simulink model "fw_watchdog_mgr"  (R2026b)
settings: Solver=VariableStepAuto
undefined symbols (not defined in the file or in its folder): DiscIntNeverNeededParam, P, ShaddadMode, Ts
libraries: simulink x10
settings Model: Creator=aomar  LastModifiedBy=aomar

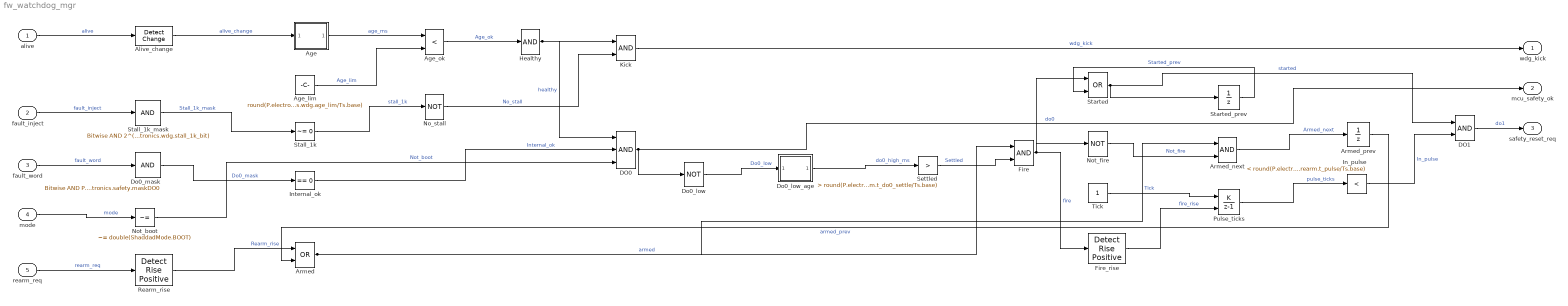
== system fw_watchdog_mgr ==
  alive : Inport  OutDataTypeStr=uint8  PortDimensions=3  SampleTime=Ts.base
  fault_inject : Inport  Port=2  OutDataTypeStr=uint32  SampleTime=Ts.base
  fault_word : Inport  Port=3  OutDataTypeStr=uint32  SampleTime=Ts.base
  mode : Inport  Port=4  OutDataTypeStr=uint8  SampleTime=Ts.base
  rearm_req : Inport  Port=5  OutDataTypeStr=boolean  SampleTime=Ts.base
  Age : Subsystem
  Age_lim : Constant  Value=round(P.electronics.wdg.age_lim/Ts.base)  OutDataTypeStr=uint16  SampleTime=Ts.base
  Age_ok : RelationalOperator  Operator=<  OutDataTypeStr=boolean  RndMeth=Simplest  InputSameDT=off
  Alive_change : simulink/Logic and Bit Operations/Detect Change  vinit=0  OutDataTypeStr=boolean
  Armed : Logic  Operator=OR  AllPortsSameDT=off  OutDataTypeStr=boolean
  Armed_next : Logic  AllPortsSameDT=off  OutDataTypeStr=boolean
  Armed_prev : UnitDelay  InitialCondition=false  SampleTime=-1
  DO0 : Logic  Inputs=3  AllPortsSameDT=off  OutDataTypeStr=boolean
  DO1 : Logic  AllPortsSameDT=off  OutDataTypeStr=boolean
  Do0_low : Logic  Operator=NOT  Inputs=1  AllPortsSameDT=off  OutDataTypeStr=boolean
  Do0_low_age : Subsystem
  Do0_mask : simulink/Logic and Bit Operations/Bitwise Operator  logicop=AND  UseBitMask=on  BitMask=P.electronics.safety.maskDO0  BitMaskRealWorld=Stored Integer
  Fire : Logic  AllPortsSameDT=off  OutDataTypeStr=boolean
  Fire_rise : simulink/Logic and Bit Operations/Detect Rise Positive  vinit=0  OutDataTypeStr=boolean
  Healthy : Logic  Inputs=1  AllPortsSameDT=off  OutDataTypeStr=boolean
  In_pulse : simulink/Logic and Bit Operations/Compare To Constant  relop=<  const=round(P.electronics.safety.rearm.t_pulse/Ts.base)  OutDataTypeStr=boolean
  Internal_ok : simulink/Logic and Bit Operations/Compare To Zero  relop===  OutDataTypeStr=boolean
  Kick : Logic  AllPortsSameDT=off  OutDataTypeStr=boolean
  No_stall : Logic  Operator=NOT  Inputs=1  AllPortsSameDT=off  OutDataTypeStr=boolean
  Not_boot : simulink/Logic and Bit Operations/Compare To Constant  relop=~=  const=double(ShaddadMode.BOOT)  OutDataTypeStr=boolean
  Not_fire : Logic  Operator=NOT  Inputs=1  AllPortsSameDT=off  OutDataTypeStr=boolean
  Pulse_ticks : DiscreteIntegrator  IntegratorMethod=Accumulation: Forward Euler  ExternalReset=rising  SampleTime=-1  OutDataTypeStr=single  LimitOutput=on  UpperSaturationLimit=round(P.electronics.safety.rearm.t_pulse/Ts.base) + 1  LowerSaturationLimit=0  ICPrevOutput=DiscIntNeverNeededParam  ICPrevScaledInput=DiscIntNeverNeededParam
  Rearm_rise : simulink/Logic and Bit Operations/Detect Rise Positive  vinit=0  OutDataTypeStr=boolean
  Settled : simulink/Logic and Bit Operations/Compare To Constant  relop=>  const=round(P.electronics.safety.rearm.t_do0_settle/Ts.base)  OutDataTypeStr=boolean
  Stall_1k : simulink/Logic and Bit Operations/Compare To Zero  relop=~=  OutDataTypeStr=boolean
  Stall_1k_mask : simulink/Logic and Bit Operations/Bitwise Operator  logicop=AND  UseBitMask=on  BitMask=2^(P.electronics.wdg.stall_1k_bit)  BitMaskRealWorld=Stored Integer
  Started : Logic  Operator=OR  AllPortsSameDT=off  OutDataTypeStr=boolean
  Started_prev : UnitDelay  InitialCondition=false  SampleTime=-1
  Tick : Constant  OutDataTypeStr=single  SampleTime=Ts.base
  wdg_kick : Outport  OutDataTypeStr=boolean
  mcu_safety_ok : Outport  Port=2  OutDataTypeStr=boolean
  safety_reset_req : Outport  Port=3  OutDataTypeStr=boolean
  wires:
  alive/1 -> Alive_change/1  "alive"
  fault_inject/1 -> Stall_1k_mask/1  "fault_inject"
  fault_word/1 -> Do0_mask/1  "fault_word"
  mode/1 -> Not_boot/1  "mode"
  rearm_req/1 -> Rearm_rise/1  "rearm_req"
  Not_boot/1 -> DO0/3  "Not_boot"
  Stall_1k_mask/1 -> Stall_1k/1  "Stall_1k_mask"
  Do0_mask/1 -> Internal_ok/1  "Do0_mask"
  Alive_change/1 -> Age/1(fresh)  "alive_change"
  Rearm_rise/1 -> Armed/1  "Rearm_rise"
  Age_lim/1 -> Age_ok/2  "Age_lim"
  Stall_1k/1 -> No_stall/1  "stall_1k"
  Internal_ok/1 -> DO0/2  "Internal_ok"
  Armed/1 -> Armed_next/1, Fire/1  "armed"
  Age/1(ticks) -> Age_ok/1  "age_ms"
  Age_ok/1 -> Healthy/1  "Age_ok"
  No_stall/1 -> Kick/2  "No_stall"
  Healthy/1 -> DO0/1, Kick/1  "healthy"
  Kick/1 -> wdg_kick/1  "wdg_kick"
  DO0/1 -> mcu_safety_ok/1, Do0_low/1  "do0"
  Do0_low/1 -> Do0_low_age/1(fresh)  "Do0_low"
  Do0_low_age/1(ticks) -> Settled/1  "do0_high_ms"
  Settled/1 -> Fire/2  "Settled"
  Fire/1 -> Fire_rise/1, Started/1, Not_fire/1  "fire"
  Started/1 -> DO1/1, Started_prev/1  "started"
  Not_fire/1 -> Armed_next/2  "Not_fire"
  Tick/1 -> Pulse_ticks/1  "Tick"
  Fire_rise/1 -> Pulse_ticks/2  "fire_rise"
  Armed_next/1 -> Armed_prev/1  "Armed_next"
  Started_prev/1 -> Started/2  "Started_prev"
  Pulse_ticks/1 -> In_pulse/1  "pulse_ticks"
  In_pulse/1 -> DO1/2  "In_pulse"
  Armed_prev/1 -> Armed/2  "armed_prev"
  DO1/1 -> safety_reset_req/1  "do1"

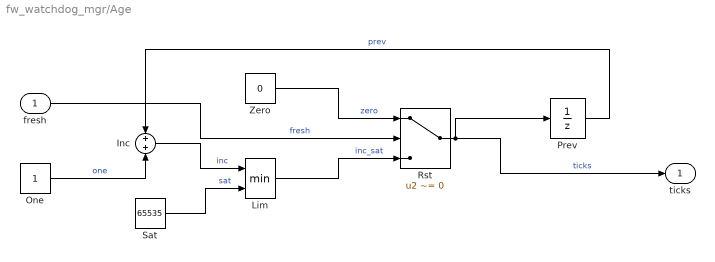
== system fw_watchdog_mgr/Age ==
  fresh : Inport
  Inc : Sum  OutDataTypeStr=uint16  SaturateOnIntegerOverflow=on
  Lim : MinMax  Inputs=2
  One : Constant  OutDataTypeStr=uint16  SampleTime=-1
  Prev : UnitDelay  SampleTime=-1
  Rst : Switch  Criteria=u2 ~= 0  SaturateOnIntegerOverflow=off  InputSameDT=off
  Sat : Constant  Value=65535  OutDataTypeStr=uint16  SampleTime=-1
  Zero : Constant  Value=0  OutDataTypeStr=uint16  SampleTime=-1
  ticks : Outport
  wires:
  fresh/1 -> Rst/2  "fresh"
  One/1 -> Inc/2  "one"
  Inc/1 -> Lim/1  "inc"
  Sat/1 -> Lim/2  "sat"
  Zero/1 -> Rst/1  "zero"
  Lim/1 -> Rst/3  "inc_sat"
  Rst/1 -> ticks/1, Prev/1  "ticks"
  Prev/1 -> Inc/1  "prev"

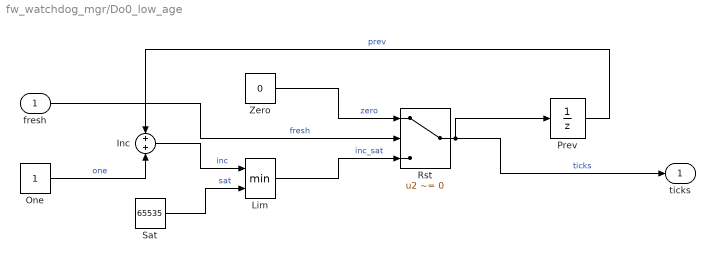
== system fw_watchdog_mgr/Do0_low_age ==
  fresh : Inport
  Inc : Sum  OutDataTypeStr=uint16  SaturateOnIntegerOverflow=on
  Lim : MinMax  Inputs=2
  One : Constant  OutDataTypeStr=uint16  SampleTime=-1
  Prev : UnitDelay  SampleTime=-1
  Rst : Switch  Criteria=u2 ~= 0  SaturateOnIntegerOverflow=off  InputSameDT=off
  Sat : Constant  Value=65535  OutDataTypeStr=uint16  SampleTime=-1
  Zero : Constant  Value=0  OutDataTypeStr=uint16  SampleTime=-1
  ticks : Outport
  wires:
  fresh/1 -> Rst/2  "fresh"
  One/1 -> Inc/2  "one"
  Inc/1 -> Lim/1  "inc"
  Sat/1 -> Lim/2  "sat"
  Zero/1 -> Rst/1  "zero"
  Lim/1 -> Rst/3  "inc_sat"
  Rst/1 -> ticks/1, Prev/1  "ticks"
  Prev/1 -> Inc/1  "prev"
